simulink model "Vector_control_FOC_with_SVPWM_of_3_phase_induction_motor_drive"  (R2024a)
settings: Solver=ode4  StartTime=0.0  StopTime=3  FixedStep=Ts  MaxStep=1e-4  RelTol=1e-3
PreLoadFcn:
  | Ts=1e-5;
InitFcn:
  | Ts=1e-5;
undefined symbols (not defined in the file): DiscIntNeverNeededParam
libraries: slpidlib x3, spsUniversalBridgeLib x1, spsDCVoltageSourceLib x1, powerlib_extras x1, spsAsynchronousMachineSIUnitsLib x1, simulink x1, spsVoltageMeasurementLib x1, spspowerguiLib x1
Description:
  | Copyright 2011-2013 Ruan Jiayang, Tsinghua Univ.
settings Model: Creator=Hoang Lehuy, Laval University  LastModifiedBy=haris
settings SolverCC: AlgebraicLoopSolver=TrustRegion
settings DataIOCC: SaveFinalState=on  SaveFormat=Array  SignalLoggingSaveFormat=ModelDataLogs  SaveOutput=off  SaveTime=off  ReturnWorkspaceOutputs=off  SignalLoggingName=sigsOut
settings OptimizationCC: BlockReduction=off  ExpressionDepthLimit=2147483647  InitFltsAndDblsToZero=on  LifeSpan=inf
settings DebuggingCC: SaveWithParameterizedLinksMsg=none  UnderspecifiedInitializationDetection=Classic  MergeDetectMultiDrivingBlocksExec=none  CheckExecutionContextPreStartOutputMsg=on  SignalResolutionControl=TryResolveAllWithWarning  MultiTaskDSMMsg=warning  MultiTaskCondExecSysMsg=none  FcnCallInpInsideContextMsg=warning  UnconnectedInputMsg=warning  UnconnectedLineMsg=warning  StateNameClashWarn=warning  SFUnexpectedBacktrackingDiag=warning  SFNoUnconditionalDefaultTransitionDiag=warning  SFExecutionAtInitializationDiag=none  ArithmeticOperatorsInVariantConditions=warning
settings HardwareCC: ProdBitPerPointer=32  ProdBitPerSizeT=32  ProdBitPerPtrDiffT=32  ProdLargestAtomicFloat=None  ProdIntDivRoundTo=Undefined  ProdEndianess=Unspecified  ProdWordSize=32  ProdHWDeviceType=32-bit Generic  TargetUnknown=on
settings ModelReferenceCC: PropagateSignalLabelsOutOfModel=off
settings SFSimCC: SimUseLocalCustomCode=off  SimParseCustomCode=off  CustomCodeUndefinedFunction=UseInterfaceOnly
settings RTWCC: RTWUseLocalCustomCode=off  GPUComputeCapability=3.5
settings CodeAppCC: StateflowObjectComments=on
settings GRTTargetCC: TargetFcnLib=ansi_tfl_tmw.mat  TargetLangStandard=C89/C90 (ANSI)  CombineOutputUpdateFcns=off  GRTInterface=on
settings ConfigComp: CovMetricSettings=dw  CovSaveCumulativeToWorkspaceVar=on  CovSaveSingleToWorkspaceVar=on  CovExternalEMLEnable=off

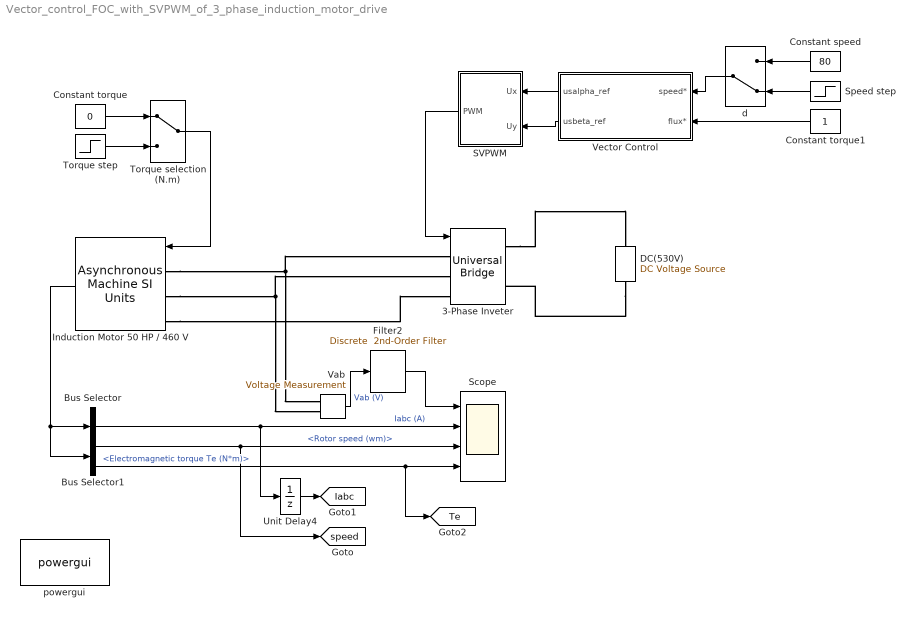
== system Vector_control_FOC_with_SVPWM_of_3_phase_induction_motor_drive ==
  3-Phase Inveter : spsUniversalBridgeLib/Universal Bridge  Arms=3  SnubberResistance=1e5  SnubberCapacitance=1e-6  Device=IGBT / Diodes  Ron=1e-3  Lon=0  ForwardVoltages="[1.1  0.75]"  ForwardVoltage=0  GTOparameters=[ 10e-6 , 20e-6 ]  IGBTparameters=[ 1e-6 , 2e-6 ]  Measurements=None  Measurements_2=None  converterType=Rectifier
  Bus Selector : BusSelector  OutputSignals=Stator measurements.Stator current is_a (A),Stator measurements.Stator current is_b (A),Stator measurements.Stator current is_c (A)  OutputAsBus=on
  Bus Selector1 : BusSelector  OutputSignals=Mechanical.Rotor speed (wm),Mechanical.Electromagnetic torque Te (N*m)
  Constant speed : Constant  Value=80
  Constant torque : Constant  Value=0
  Constant torque1 : Constant
  DC(530V) : spsDCVoltageSourceLib/DC Voltage Source  Amplitude=530  Measurements=None
  Filter2 : powerlib_extras/Discrete  Control Blocks/Discrete  2nd-Order Filter  FilterType=Lowpass  Fo=100  Zeta=0.707  Ts=Ts  Initialize=off  Vac_Init=[0.8 -25 60]  Vdc_Init=-0.4  PlotResponse=off  param1=[1 500 1]
  Induction Motor 50 HP / 460 V : spsAsynchronousMachineSIUnitsLib/Asynchronous Machine SI Units  RotorType=Squirrel-cage  PresetModel=No  MechanicalLoad=Torque Tm  ShowDetailedParameters=on  ReferenceFrame=Stationary  Units=SI  MeasurementBus=off  NominalParameters=[ 50*746, 460, 60 ]  VoltageRatio=1  Stator=[ 0.087 0.8e-3 ]  Rotor="[ 0.228  0.8e-3 ]"  Cage1=[0.4155 0.002066]  Cage2=[0.4168 0.0003495]  Lm=34.7e-3  Mechanical="[1.662  0.01 2 ]"  PolePairs=2  InitialConditions="[ 1, 0 ,  0 , 0 , 0 , 0 , 0 , 0 ]"  SimulateSaturation=off  Saturation=[0 0;0 0]  LoadFlowParameters=0  TsPowergui=0  TsBlock=-1  IterativeModel=Trapezoidal non iterative  IterativeDiscreteModel=Trapezoidal non iterative  Pmec=1.492e+006
      settings: AttributesFormatString=\n
  SVPWM : Subsystem
  Scope : Scope  NumInputPorts=4
  Speed step : Step  Time=1.5  Before=80  After=160  SampleTime=Ts
  Torque selection (N.m) : ManualSwitch
  Torque step : Step  Time=1.8  After=200  SampleTime=0
  Unit Delay4 : UnitDelay  SampleTime=Ts
  Vab : spsVoltageMeasurementLib/Voltage Measurement  Tag=PoWeRsYsTeMmEaSuReMeNt  PhasorSimulation=off  OutputType=Magnitude  PSBequivalent=0
  Vector Control : Subsystem
  d : ManualSwitch  CurrentSetting=0
  powergui : spspowerguiLib/powergui  Priority=2  SimulationMode=Continuous  SampleTime=Ts  frequency=60  Iterations=50  frequencyindice=0  Pbase=100e6  ErrMax=1e-4  UnitsV=kV  UnitsW=MW  buscounter=0  FunctionMessages=off  echomessages=off  EnableUseOfTLC=off  CurrentSourceSwitches=off  DisableSnubberDevices=off  DisableRonSwitches=off  DisableVfSwitches=off  DisplayEquations=off  AutomaticDiscreteSolvers=off  SolverType=Tustin/Backward Euler (TBE)  Interpol=off  ExternalGateDelay=off  methode=off  Ts=0  x0status=blocks  SPID=off  SwTol=0  HookPort=off  NonlinearTolerance=1e-4  nMaxIteration=100  ContinueOnMaxIteration=off  RestoreLinks=warning  ResistiveCurrentMeasurement=off  Frange=[0:2:500]  Ylog=off  Xlog=on  ShowGrid=off  save=off  variable=ZData  structure=0  ZoomFFT=on  StartTime=0.0  cycles=1  DisplayStyle=off  fundamental=60  FreqAxis=off  MaxFrequency=1000  frequencyindicesteady=1  RmsSteady=1  display=off
  tag scope: Iabc=global, Te=global, speed=global
  wires:
  Bus Selector1/1 -> Scope/3, [speed]  "<Rotor speed (wm)>"
  Torque step/1 -> Torque selection (N.m)/2
  Constant torque/1 -> Torque selection (N.m)/1
  Constant speed/1 -> d/1
  Speed step/1 -> d/2
  Bus Selector/1 -> Scope/2, Unit Delay4/1  "Iabc (A)"
  Bus Selector1/2 -> Scope/4, [Te]  "<Electromagnetic torque Te (N*m)>"
  Torque selection (N.m)/1 -> Induction Motor 50 HP / 460 V/1
  Induction Motor 50 HP / 460 V/1 -> Bus Selector1/1, Bus Selector/1
  Unit Delay4/1 -> [Iabc]
  d/1 -> Vector Control/1(speed*)
  Constant torque1/1 -> Vector Control/2(flux*)
  Vector Control/1(usalpha_ref) -> SVPWM/1(Ux)
  Vector Control/2(usbeta_ref) -> SVPWM/2(Uy)
  SVPWM/1(PWM) -> 3-Phase Inveter/1
  Vab/1 -> Filter2/1  "Vab (V)"
  Filter2/1 -> Scope/1
  connections:
  Induction Motor 50 HP / 460 V/LConn2 -- Vab/LConn2 -- 3-Phase Inveter/LConn2
  Induction Motor 50 HP / 460 V/LConn1 -- Vab/LConn1 -- 3-Phase Inveter/LConn1
  Induction Motor 50 HP / 460 V/LConn3 -- 3-Phase Inveter/LConn3
  3-Phase Inveter/RConn1 -- DC(530V)/RConn1
  DC(530V)/LConn1 -- 3-Phase Inveter/RConn2

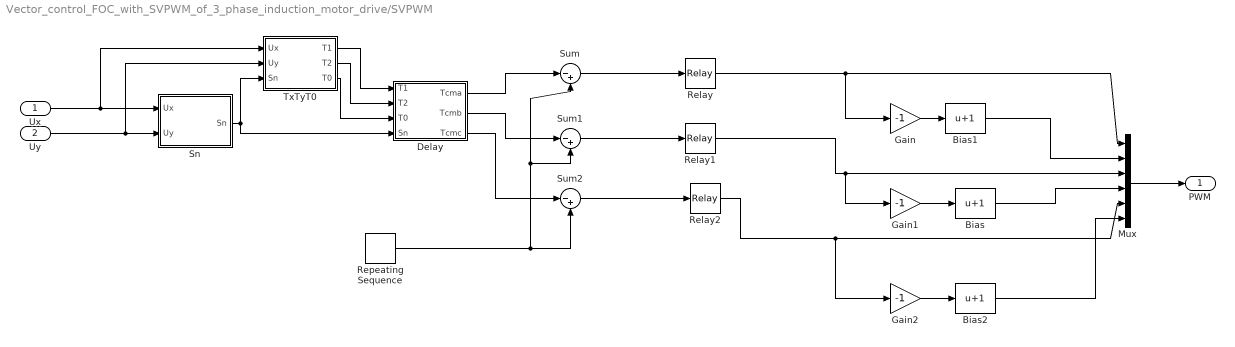
== system Vector_control_FOC_with_SVPWM_of_3_phase_induction_motor_drive/SVPWM ==
  Ux : Inport
  Uy : Inport  Port=2
  Bias : Bias  Bias=1  SaturateOnIntegerOverflow=off
  Bias1 : Bias  Bias=1  SaturateOnIntegerOverflow=off
  Bias2 : Bias  Bias=1  SaturateOnIntegerOverflow=off
  Delay : MATLAB Function  TreatAsAtomicUnit=on
  Gain : Gain  Gain=-1
  Gain1 : Gain  Gain=-1
  Gain2 : Gain  Gain=-1
  Mux : Mux  Inputs=6
  Relay : Relay  OnSwitchValue=0  OffSwitchValue=0
  Relay1 : Relay  OnSwitchValue=0  OffSwitchValue=0
  Relay2 : Relay  OnSwitchValue=0  OffSwitchValue=0
  Repeating Sequence : simulink/Sources/Repeating Sequence  rep_seq_t=[0 1/2000/2 1/2000]  rep_seq_y=[0 1/2000/2 0]
  Sn : MATLAB Function  TreatAsAtomicUnit=on
  Sum : Sum  Inputs=|-+
  Sum1 : Sum  Inputs=|-+
  Sum2 : Sum  Inputs=|-+
  TxTyT0 : MATLAB Function  TreatAsAtomicUnit=on
  PWM : Outport
  wires:
  Delay/1(Tcma) -> Sum/1
  Delay/2(Tcmb) -> Sum1/1
  Delay/3(Tcmc) -> Sum2/1
  Repeating Sequence/1 -> Sum/2, Sum1/2, Sum2/2
  Sum/1 -> Relay/1
  Sum2/1 -> Relay2/1
  Sum1/1 -> Relay1/1
  Relay1/1 -> Mux/3, Gain1/1
  Relay2/1 -> Mux/5, Gain2/1
  Sn/1(Sn) -> TxTyT0/3(Sn), Delay/4(Sn)
  TxTyT0/1(T1) -> Delay/1(T1)
  TxTyT0/2(T2) -> Delay/2(T2)
  TxTyT0/3(T0) -> Delay/3(T0)
  Mux/1 -> PWM/1
  Gain1/1 -> Bias/1
  Gain/1 -> Bias1/1
  Gain2/1 -> Bias2/1
  Bias1/1 -> Mux/2
  Bias/1 -> Mux/4
  Bias2/1 -> Mux/6
  Relay/1 -> Mux/1, Gain/1
  Ux/1 -> Sn/1(Ux), TxTyT0/1(Ux)
  Uy/1 -> Sn/2(Uy), TxTyT0/2(Uy)

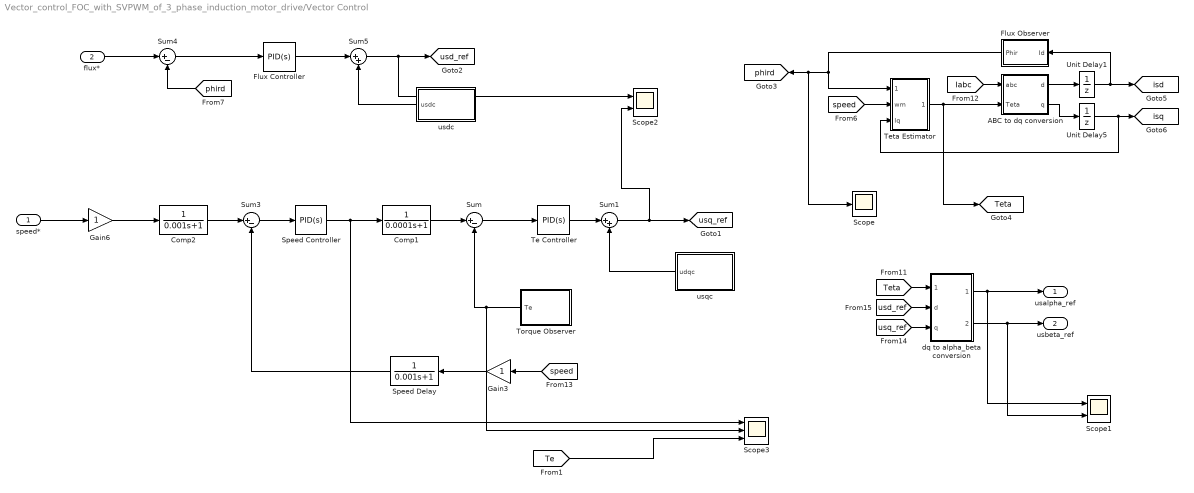
== system Vector_control_FOC_with_SVPWM_of_3_phase_induction_motor_drive/Vector Control ==
  speed* : Inport
  flux* : Inport  Port=2
  ABC to dq conversion : Subsystem
  Comp1 : TransferFcn  Denominator=[0.0001 1]
  Comp2 : TransferFcn  Denominator=[0.001 1]
  Flux Controller : slpidlib/PID Controller  Controller=PID  Form=Parallel  TimeDomain=Continuous-time  UseExternalTs=off  SampleTime=1  IntegratorMethod=Forward Euler  FilterMethod=Forward Euler  ControllerParametersSource=internal  P=138.2107  I=247.3835  UseKiTs=off  D=0  UseExternalDerivativeSource=off  N=100  UseFilter=on  TunerSelectOption=Transfer Function Based (PID Tuner App)  InitialConditionSource=internal  InitialConditionForIntegrator=100  InitialConditionForFilter=0  DifferentiatorICPrevScaledInput=0  ExternalReset=none  TrackingMode=off  Kt=1  LimitOutput=on  SatLimitsSource=internal  UpperSaturationLimit=200  LowerSaturationLimit=-200  LinearizeAsGain=off  AntiWindupMode=clamping  Kb=1  LimitIntegrator=off  UpperIntegratorSaturationLimit=inf  LowerIntegratorSaturationLimit=-inf  POutMin=[]  POutMax=[]  IOutMin=[]  IOutMax=[]  DOutMin=[]  DOutMax=[]  NOutMin=[]  NOutMax=[]  SumOutMin=[]  SumOutMax=[]  SaturationOutMin=[]  SaturationOutMax=[]  PParamMin=[]  PParamMax=[]  IParamMin=[]  IParamMax=[]  DParamMin=[]  DParamMax=[]  NParamMin=[]  NParamMax=[]  KbParamMin=[]  KbParamMax=[]  KtParamMin=[]  KtParamMax=[]  KbOutMin=[]  KbOutMax=[]  KtOutMin=[]  KtOutMax=[]  IntegratorOutMin=[]  IntegratorOutMax=[]  FilterOutMin=[]  FilterOutMax=[]  SumI1OutMin=[]  SumI1OutMax=[]  SumI2OutMin=[]  SumI2OutMax=[]  SumI3OutMin=[]  SumI3OutMax=[]  SumI4OutMin=[]  SumI4OutMax=[]  SumDOutMin=[]  SumDOutMax=[]  DifferentiatorOutMin=[]  DifferentiatorOutMax=[]  FilterDiffOutCoefMin=[]  FilterDiffOutCoefMax=[]  ReciprocalOutMin=[]  ReciprocalOutMax=[]  SumDenOutMin=[]  SumDenOutMax=[]  SumNumOutMin=[]  SumNumOutMax=[]  DivideOutMin=[]  DivideOutMax=[]  UdiffTsProdOutMin=[]  UdiffTsProdOutMax=[]  NTsProdOutMin=[]  NTsProdOutMax=[]  UintegralTsProdOutMin=[]  UintegralTsProdOutMax=[]  UngainTsProdOutMin=[]  UngainTsProdOutMax=[]  ClampingZeroOutDataTypeStr=Inherit: Inherit via back propagation  ClampingZeroOutMin=[]  ClampingZeroOutMax=[]  FilterDenConstantOutDataTypeStr=Inherit: Inherit via back propagation  FilterDenConstantOutMin=[]  FilterDenConstantOutMax=[]  PCopyOutDataTypeStr=Inherit: Inherit via back propagation  PCopyOutMin=[]  PCopyOutMax=[]  NCopyOutDataTypeStr=Inherit: Inherit via back propagation  NCopyOutMin=[]  NCopyOutMax=[]  IntegratorContinuousStateAttributes=''  IntegratorStateMustResolveToSignalObject=off  IntegratorRTWStateStorageClass=Auto  FilterContinuousStateAttributes=''  FilterStateMustResolveToSignalObject=off  FilterRTWStateStorageClass=Auto  ParallelPVariant=InternalParameters  IdealPVariant=Disabled  IVariant=InternalParameters  DVariant=InternalParameters  IntegratorVariant=Continuous  SatVariant=Enabled  AWVariant=ContClampingParallel  PCopyVariant=Disabled  TRVariant=Disabled  FdbkBlocksVariant=Forward  IdealPFdbkVariant=Disabled  SatFdbkVariant=Disabled  DerivativeFilterVariant=ContFilter  NVariant=InternalParameters  NCopyVariant=Disabled  FilterICVariant=InternalICsFilter  IntegratorICVariant=InternalICs  ExternalResetVariant=Disabled  TRSumVariant=Passthrough  SumFdbkVariant=Disabled  SumVariant=Sum_PID  TsampFilterVariant=InternalTs  TsampNgainVariant=Passthrough  TsampIntegralVariant=Disabled_SignalSpec  ExternalSaturationOutDataTypeStr=Inherit: Same as second input  DerivativeSourceVariant=ErrorSignal
  Flux Observer : Subsystem  mask(Flux Calcultation){}
      mask init:
      | NF=0.44572610323020e-6;
      | DF=[1 -0.99998715486734];
  Gain3 : Gain
  Gain6 : Gain
  Scope : Scope
  Scope1 : Scope  NumInputPorts=2
  Scope2 : Scope  NumInputPorts=2
  Scope3 : Scope  NumInputPorts=3
  Speed Controller : slpidlib/PID Controller  Controller=PID  Form=Parallel  TimeDomain=Continuous-time  UseExternalTs=off  SampleTime=1  IntegratorMethod=Forward Euler  FilterMethod=Forward Euler  ControllerParametersSource=internal  P=166.2  I=27700  UseKiTs=off  D=0  UseExternalDerivativeSource=off  N=100  UseFilter=on  TunerSelectOption=Transfer Function Based (PID Tuner App)  InitialConditionSource=internal  InitialConditionForIntegrator=50  InitialConditionForFilter=0  DifferentiatorICPrevScaledInput=0  ExternalReset=none  TrackingMode=off  Kt=1  LimitOutput=on  SatLimitsSource=internal  UpperSaturationLimit=200  LowerSaturationLimit=-200  LinearizeAsGain=off  AntiWindupMode=clamping  Kb=1  LimitIntegrator=off  UpperIntegratorSaturationLimit=inf  LowerIntegratorSaturationLimit=-inf  POutMin=[]  POutMax=[]  IOutMin=[]  IOutMax=[]  DOutMin=[]  DOutMax=[]  NOutMin=[]  NOutMax=[]  SumOutMin=[]  SumOutMax=[]  SaturationOutMin=[]  SaturationOutMax=[]  PParamMin=[]  PParamMax=[]  IParamMin=[]  IParamMax=[]  DParamMin=[]  DParamMax=[]  NParamMin=[]  NParamMax=[]  KbParamMin=[]  KbParamMax=[]  KtParamMin=[]  KtParamMax=[]  KbOutMin=[]  KbOutMax=[]  KtOutMin=[]  KtOutMax=[]  IntegratorOutMin=[]  IntegratorOutMax=[]  FilterOutMin=[]  FilterOutMax=[]  SumI1OutMin=[]  SumI1OutMax=[]  SumI2OutMin=[]  SumI2OutMax=[]  SumI3OutMin=[]  SumI3OutMax=[]  SumI4OutMin=[]  SumI4OutMax=[]  SumDOutMin=[]  SumDOutMax=[]  DifferentiatorOutMin=[]  DifferentiatorOutMax=[]  FilterDiffOutCoefMin=[]  FilterDiffOutCoefMax=[]  ReciprocalOutMin=[]  ReciprocalOutMax=[]  SumDenOutMin=[]  SumDenOutMax=[]  SumNumOutMin=[]  SumNumOutMax=[]  DivideOutMin=[]  DivideOutMax=[]  UdiffTsProdOutMin=[]  UdiffTsProdOutMax=[]  NTsProdOutMin=[]  NTsProdOutMax=[]  UintegralTsProdOutMin=[]  UintegralTsProdOutMax=[]  UngainTsProdOutMin=[]  UngainTsProdOutMax=[]  ClampingZeroOutDataTypeStr=Inherit: Inherit via back propagation  ClampingZeroOutMin=[]  ClampingZeroOutMax=[]  FilterDenConstantOutDataTypeStr=Inherit: Inherit via back propagation  FilterDenConstantOutMin=[]  FilterDenConstantOutMax=[]  PCopyOutDataTypeStr=Inherit: Inherit via back propagation  PCopyOutMin=[]  PCopyOutMax=[]  NCopyOutDataTypeStr=Inherit: Inherit via back propagation  NCopyOutMin=[]  NCopyOutMax=[]  IntegratorContinuousStateAttributes=''  IntegratorStateMustResolveToSignalObject=off  IntegratorRTWStateStorageClass=Auto  FilterContinuousStateAttributes=''  FilterStateMustResolveToSignalObject=off  FilterRTWStateStorageClass=Auto  ParallelPVariant=InternalParameters  IdealPVariant=Disabled  IVariant=InternalParameters  DVariant=InternalParameters  IntegratorVariant=Continuous  SatVariant=Enabled  AWVariant=ContClampingParallel  PCopyVariant=Disabled  TRVariant=Disabled  FdbkBlocksVariant=Forward  IdealPFdbkVariant=Disabled  SatFdbkVariant=Disabled  DerivativeFilterVariant=ContFilter  NVariant=InternalParameters  NCopyVariant=Disabled  FilterICVariant=InternalICsFilter  IntegratorICVariant=InternalICs  ExternalResetVariant=Disabled  TRSumVariant=Passthrough  SumFdbkVariant=Disabled  SumVariant=Sum_PID  TsampFilterVariant=InternalTs  TsampNgainVariant=Passthrough  TsampIntegralVariant=Disabled_SignalSpec  ExternalSaturationOutDataTypeStr=Inherit: Same as second input  DerivativeSourceVariant=ErrorSignal
  Speed Delay : TransferFcn  Denominator=[0.001 1]
  Sum : Sum  Inputs=|+-
  Sum1 : Sum  Inputs=|++
  Sum3 : Sum  Inputs=|+-
  Sum4 : Sum  Inputs=|+-
  Sum5 : Sum  Inputs=|++
  Te Controller : slpidlib/PID Controller  Controller=PID  Form=Parallel  TimeDomain=Continuous-time  UseExternalTs=off  SampleTime=1  IntegratorMethod=Forward Euler  FilterMethod=Forward Euler  ControllerParametersSource=internal  P=2.69732  I=148.34534  UseKiTs=off  D=0  UseExternalDerivativeSource=off  N=100  UseFilter=on  TunerSelectOption=Transfer Function Based (PID Tuner App)  InitialConditionSource=internal  InitialConditionForIntegrator=100  InitialConditionForFilter=0  DifferentiatorICPrevScaledInput=0  ExternalReset=none  TrackingMode=off  Kt=1  LimitOutput=on  SatLimitsSource=internal  UpperSaturationLimit=200  LowerSaturationLimit=-200  LinearizeAsGain=off  AntiWindupMode=clamping  Kb=1  LimitIntegrator=off  UpperIntegratorSaturationLimit=inf  LowerIntegratorSaturationLimit=-inf  POutMin=[]  POutMax=[]  IOutMin=[]  IOutMax=[]  DOutMin=[]  DOutMax=[]  NOutMin=[]  NOutMax=[]  SumOutMin=[]  SumOutMax=[]  SaturationOutMin=[]  SaturationOutMax=[]  PParamMin=[]  PParamMax=[]  IParamMin=[]  IParamMax=[]  DParamMin=[]  DParamMax=[]  NParamMin=[]  NParamMax=[]  KbParamMin=[]  KbParamMax=[]  KtParamMin=[]  KtParamMax=[]  KbOutMin=[]  KbOutMax=[]  KtOutMin=[]  KtOutMax=[]  IntegratorOutMin=[]  IntegratorOutMax=[]  FilterOutMin=[]  FilterOutMax=[]  SumI1OutMin=[]  SumI1OutMax=[]  SumI2OutMin=[]  SumI2OutMax=[]  SumI3OutMin=[]  SumI3OutMax=[]  SumI4OutMin=[]  SumI4OutMax=[]  SumDOutMin=[]  SumDOutMax=[]  DifferentiatorOutMin=[]  DifferentiatorOutMax=[]  FilterDiffOutCoefMin=[]  FilterDiffOutCoefMax=[]  ReciprocalOutMin=[]  ReciprocalOutMax=[]  SumDenOutMin=[]  SumDenOutMax=[]  SumNumOutMin=[]  SumNumOutMax=[]  DivideOutMin=[]  DivideOutMax=[]  UdiffTsProdOutMin=[]  UdiffTsProdOutMax=[]  NTsProdOutMin=[]  NTsProdOutMax=[]  UintegralTsProdOutMin=[]  UintegralTsProdOutMax=[]  UngainTsProdOutMin=[]  UngainTsProdOutMax=[]  ClampingZeroOutDataTypeStr=Inherit: Inherit via back propagation  ClampingZeroOutMin=[]  ClampingZeroOutMax=[]  FilterDenConstantOutDataTypeStr=Inherit: Inherit via back propagation  FilterDenConstantOutMin=[]  FilterDenConstantOutMax=[]  PCopyOutDataTypeStr=Inherit: Inherit via back propagation  PCopyOutMin=[]  PCopyOutMax=[]  NCopyOutDataTypeStr=Inherit: Inherit via back propagation  NCopyOutMin=[]  NCopyOutMax=[]  IntegratorContinuousStateAttributes=''  IntegratorStateMustResolveToSignalObject=off  IntegratorRTWStateStorageClass=Auto  FilterContinuousStateAttributes=''  FilterStateMustResolveToSignalObject=off  FilterRTWStateStorageClass=Auto  ParallelPVariant=InternalParameters  IdealPVariant=Disabled  IVariant=InternalParameters  DVariant=InternalParameters  IntegratorVariant=Continuous  SatVariant=Enabled  AWVariant=ContClampingParallel  PCopyVariant=Disabled  TRVariant=Disabled  FdbkBlocksVariant=Forward  IdealPFdbkVariant=Disabled  SatFdbkVariant=Disabled  DerivativeFilterVariant=ContFilter  NVariant=InternalParameters  NCopyVariant=Disabled  FilterICVariant=InternalICsFilter  IntegratorICVariant=InternalICs  ExternalResetVariant=Disabled  TRSumVariant=Passthrough  SumFdbkVariant=Disabled  SumVariant=Sum_PID  TsampFilterVariant=InternalTs  TsampNgainVariant=Passthrough  TsampIntegralVariant=Disabled_SignalSpec  ExternalSaturationOutDataTypeStr=Inherit: Same as second input  DerivativeSourceVariant=ErrorSignal
  Teta Estimator : Subsystem
  Torque Observer : Subsystem
  Unit Delay1 : UnitDelay  SampleTime=Ts
  Unit Delay5 : UnitDelay  SampleTime=Ts
  dq to alpha_beta conversion : Subsystem
  usdc : Subsystem
  usqc : Subsystem
  usalpha_ref : Outport
  usbeta_ref : Outport  Port=2
  tag scope: Teta=global, isd=global, isq=global, phird=global, usd_ref=global, usq_ref=global
  wires:
  Sum/1 -> Te Controller/1
  Comp1/1 -> Sum/1
  Te Controller/1 -> Sum1/1
  usqc/1(udqc) -> Sum1/2
  Torque Observer/1(Te) -> Sum/2, Scope3/2
  Sum1/1 -> [usq_ref], Scope2/2
  [speed] -> Gain3/1
  Sum3/1 -> Speed Controller/1
  Gain3/1 -> Speed Delay/1
  Comp2/1 -> Sum3/1
  flux*/1 -> Sum4/1
  [phird] -> Sum4/2
  Sum4/1 -> Flux Controller/1
  Flux Controller/1 -> Sum5/1
  Sum5/1 -> [usd_ref], Scope2/1
  Flux Observer/1(Phir) -> Teta Estimator/1(Phird), [phird], Scope/1
  Teta Estimator/1(Teta) -> ABC to dq conversion/2(Teta), [Teta]
  [speed] -> Teta Estimator/2(wm)
  [Iabc] -> ABC to dq conversion/1(abc)
  [Teta] -> dq to alpha_beta conversion/1(Teta)
  Gain6/1 -> Comp2/1
  speed*/1 -> Gain6/1
  ABC to dq conversion/1(d) -> Unit Delay1/1
  Unit Delay1/1 -> [isd], Flux Observer/1(Id)
  ABC to dq conversion/2(q) -> Unit Delay5/1
  Unit Delay5/1 -> Teta Estimator/3(Iq), [isq]
  [usd_ref] -> dq to alpha_beta conversion/2(d)
  [usq_ref] -> dq to alpha_beta conversion/3(q)
  usdc/1(usdc) -> Sum5/2
  Speed Delay/1 -> Sum3/2
  Speed Controller/1 -> Comp1/1, Scope3/1
  [Te] -> Scope3/3
  dq to alpha_beta conversion/1(usalpha) -> usalpha_ref/1, Scope1/1
  dq to alpha_beta conversion/2(usbeta) -> usbeta_ref/1, Scope1/2

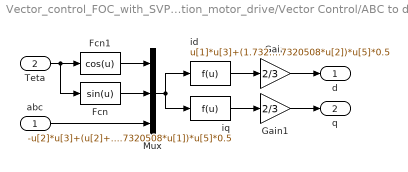
== system Vector_control_FOC_with_SVPWM_of_3_phase_induction_motor_drive/Vector Control/ABC to dq conversion ==
  abc : Inport
  Teta : Inport  Port=2
  Fcn : Fcn  Expr=sin(u)
  Fcn1 : Fcn  Expr=cos(u)
  Gain : Gain  Gain=2/3  SaturateOnIntegerOverflow=on  OutDataTypeStr=Inherit: Same as input  ParamDataTypeStr=Inherit: Same as input
  Gain1 : Gain  Gain=2/3  SaturateOnIntegerOverflow=on  OutDataTypeStr=Inherit: Same as input  ParamDataTypeStr=Inherit: Same as input
  Mux : Mux  Inputs=[1 1 3]
  id : Fcn  Expr=u[1]*u[3]+(1.7320508*u[2]-u[1])*u[4]*0.5+(-u[1]-1.7320508*u[2])*u[5]*0.5
  iq : Fcn  Expr=-u[2]*u[3]+(u[2]+1.7320508*u[1])*u[4]*0.5+(u[2]-1.7320508*u[1])*u[5]*0.5
  d : Outport  InitialOutput=0
  q : Outport  Port=2  InitialOutput=0
  wires:
  Fcn/1 -> Mux/2
  Fcn1/1 -> Mux/1
  Teta/1 -> Fcn1/1, Fcn/1
  Mux/1 -> iq/1, id/1
  abc/1 -> Mux/3
  iq/1 -> Gain1/1
  id/1 -> Gain/1
  Gain/1 -> d/1
  Gain1/1 -> q/1

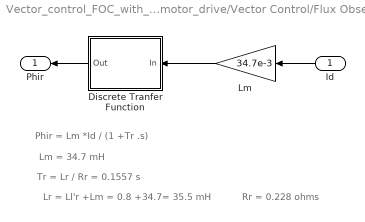
== system Vector_control_FOC_with_SVPWM_of_3_phase_induction_motor_drive/Vector Control/Flux Observer ==
  note: Phir = Lm *Id / (1 +Tr .s)
  note: Lm = 34.7 mH
  note: Lr = Ll'r +Lm = 0.8 +34.7= 35.5 mH
  note: Tr = Lr / Rr = 0.1557 s
  note: Rr = 0.228 ohms
  Id : Inport
  Discrete Tranfer Function : Subsystem  mask(First Order Low Pass Filter (Discrete)){T=0.1557, Ts=Ts}
      mask prompts: T "Time constant T (s) :"; Ts "Time step (s)"
      mask help: H(s)=1/(1+T.s)
      mask init:
      | X=[0 1 2 3 4];
      |  Y=[-2 -2 -3 -4 -4];
      |  str=sprintf('\nH=1/(1+T.s)\n T= %g s\n\n\n',T);
      | num=1;
      | den=[T 1];
      | 
      | % discrete transfer function
      | % descending powers of z
      | numd= Ts/T;
      | dend=[ 1  (Ts-T)/T];
      mask Display:
      | plot(X,Y);
      | disp(str);
  Lm : Gain  Gain=34.7e-3  SaturateOnIntegerOverflow=on  OutDataTypeStr=Inherit: Same as input  ParamDataTypeStr=Inherit: Same as input
  Phir : Outport
  wires:
  Discrete Tranfer Function/1(Out) -> Phir/1
  Id/1 -> Lm/1
  Lm/1 -> Discrete Tranfer Function/1(In)

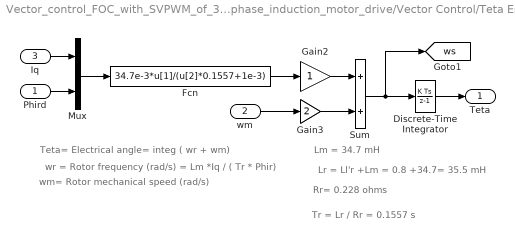
== system Vector_control_FOC_with_SVPWM_of_3_phase_induction_motor_drive/Vector Control/Teta Estimator ==
  note: Teta= Electrical angle= integ ( wr + wm)
  note: wr = Rotor frequency (rad/s) = Lm *Iq / ( Tr * Phir)
  note: Lm = 34.7 mH
  note: Rr= 0.228 ohms
  note: Lr = Ll'r +Lm = 0.8 +34.7= 35.5 mH
  note: wm= Rotor mechanical speed (rad/s)
  note: Tr = Lr / Rr = 0.1557 s
  Phird : Inport
  wm : Inport  Port=2
  Iq : Inport  Port=3
  Discrete-Time Integrator : DiscreteIntegrator  SampleTime=Ts  ICPrevOutput=DiscIntNeverNeededParam  ICPrevScaledInput=DiscIntNeverNeededParam
  Fcn : Fcn  Expr=34.7e-3*u[1]/(u[2]*0.1557+1e-3)
  Gain2 : Gain  SaturateOnIntegerOverflow=on  OutDataTypeStr=Inherit: Same as input  ParamDataTypeStr=Inherit: Same as input
  Gain3 : Gain  Gain=2  SaturateOnIntegerOverflow=on  OutDataTypeStr=Inherit: Same as input  ParamDataTypeStr=Inherit: Same as input
  Mux : Mux  Inputs=2
  Sum : Sum  InputSameDT=on  SaturateOnIntegerOverflow=on  OutDataTypeStr=Inherit: Same as first input
  Teta : Outport  InitialOutput=0
  tag scope: ws=global
  wires:
  Discrete-Time Integrator/1 -> Teta/1
  Sum/1 -> Discrete-Time Integrator/1, [ws]
  Gain3/1 -> Sum/2
  Gain2/1 -> Sum/1
  wm/1 -> Gain3/1
  Fcn/1 -> Gain2/1
  Phird/1 -> Mux/2
  Iq/1 -> Mux/1
  Mux/1 -> Fcn/1

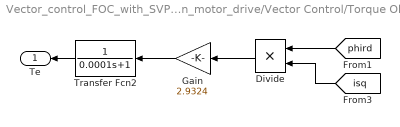
== system Vector_control_FOC_with_SVPWM_of_3_phase_induction_motor_drive/Vector Control/Torque Observer ==
  Divide : Product
  Gain : Gain  Gain=2.9324
  Transfer Fcn2 : TransferFcn  Denominator=[0.0001 1]
  Te : Outport
  wires:
  [phird] -> Divide/1
  Divide/1 -> Gain/1
  Gain/1 -> Transfer Fcn2/1
  [isq] -> Divide/2
  Transfer Fcn2/1 -> Te/1

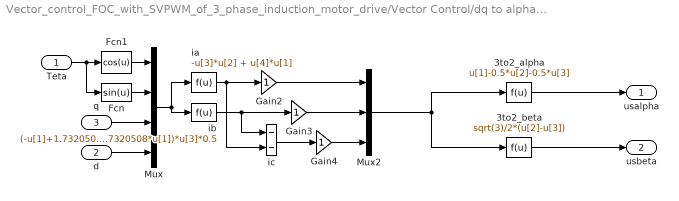
== system Vector_control_FOC_with_SVPWM_of_3_phase_induction_motor_drive/Vector Control/dq to alpha_beta conversion ==
  Teta : Inport
  d : Inport  Port=2
  q : Inport  Port=3
  3to2_alpha : Fcn  Expr=u[1]-0.5*u[2]-0.5*u[3]
  3to2_beta : Fcn  Expr=sqrt(3)/2*(u[2]-u[3])
  Fcn : Fcn  Expr=sin(u)
  Fcn1 : Fcn  Expr=cos(u)
  Gain2 : Gain  SaturateOnIntegerOverflow=on  OutDataTypeStr=Inherit: Same as input  ParamDataTypeStr=Inherit: Same as input
  Gain3 : Gain  SaturateOnIntegerOverflow=on  OutDataTypeStr=Inherit: Same as input  ParamDataTypeStr=Inherit: Same as input
  Gain4 : Gain  SaturateOnIntegerOverflow=on  OutDataTypeStr=Inherit: Same as input  ParamDataTypeStr=Inherit: Same as input
  Mux : Mux
  Mux2 : Mux  Inputs=3
  ia : Fcn  Expr=-u[3]*u[2] + u[4]*u[1]
  ib : Fcn  Expr=(-u[1]+1.7320508*u[2])*u[4]*0.5+(u[2]+1.7320508*u[1])*u[3]*0.5
  ic : Sum  Inputs=--  InputSameDT=on  SaturateOnIntegerOverflow=on  OutDataTypeStr=Inherit: Same as first input
  usalpha : Outport
  usbeta : Outport  Port=2
  wires:
  Fcn/1 -> Mux/2
  Fcn1/1 -> Mux/1
  Mux/1 -> ib/1, ia/1
  Teta/1 -> Fcn1/1, Fcn/1
  q/1 -> Mux/3
  d/1 -> Mux/4
  Gain3/1 -> Mux2/2
  ic/1 -> Gain4/1
  Gain4/1 -> Mux2/3
  Gain2/1 -> Mux2/1
  ia/1 -> Gain2/1, ic/2
  ib/1 -> Gain3/1, ic/1
  Mux2/1 -> 3to2_alpha/1, 3to2_beta/1
  3to2_alpha/1 -> usalpha/1
  3to2_beta/1 -> usbeta/1

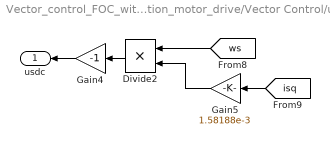
== system Vector_control_FOC_with_SVPWM_of_3_phase_induction_motor_drive/Vector Control/usdc ==
  Divide2 : Product
  Gain4 : Gain  Gain=-1
  Gain5 : Gain  Gain=1.58188e-3
  usdc : Outport
  wires:
  Divide2/1 -> Gain4/1
  [ws] -> Divide2/1
  [isq] -> Gain5/1
  Gain5/1 -> Divide2/2
  Gain4/1 -> usdc/1

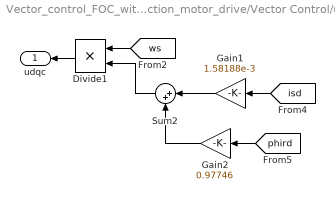
== system Vector_control_FOC_with_SVPWM_of_3_phase_induction_motor_drive/Vector Control/usqc ==
  Divide1 : Product
  Gain1 : Gain  Gain=1.58188e-3
  Gain2 : Gain  Gain=0.97746
  Sum2 : Sum  Inputs=|++
  udqc : Outport
  wires:
  [ws] -> Divide1/1
  Sum2/1 -> Divide1/2
  Gain1/1 -> Sum2/1
  Gain2/1 -> Sum2/2
  [isd] -> Gain1/1
  [phird] -> Gain2/1
  Divide1/1 -> udqc/1

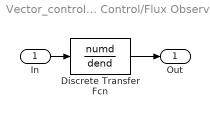
== system Vector_control_FOC_with_SVPWM_of_3_phase_induction_motor_drive/Vector Control/Flux Observer/Discrete Tranfer Function ==
  In : Inport
  Discrete Transfer Fcn : DiscreteTransferFcn  Numerator=numd  Denominator=dend  SampleTime=Ts
  Out : Outport  InitialOutput=0
  wires:
  Discrete Transfer Fcn/1 -> Out/1
  In/1 -> Discrete Transfer Fcn/1

== matlab function Vector_control_FOC_with_SVPWM_of_3_phase_induction_motor_drive/SVPWM/Sn ==
  data: Sn output; Ux input; Uy input
function Sn = S(Ux,Uy)
theta=atan2(Uy,Ux)*180/pi;
if theta>=0&&theta<60
    Sn=1;
elseif theta>=60&&theta<120
    Sn=2;
elseif theta>=120&&theta<180
    Sn=3;
elseif theta>=-180&&theta<-120
    Sn=4;
elseif theta>=-120&&theta<-60
    Sn=5;
else Sn=6;
end

== matlab function Vector_control_FOC_with_SVPWM_of_3_phase_induction_motor_drive/SVPWM/TxTyT0 ==
  data: Ux input; Uy input; Sn input; T1 output; T2 output; T0 output
function [T1,T2,T0]=T(Ux,Uy,Sn)
Ts=1/2000;
Udc=530;

X=sqrt(3)*Ts/Udc*Uy;
Y=sqrt(3)*Ts/2/Udc*(sqrt(3)*Ux+Uy);
Z=sqrt(3)*Ts/2/Udc*(-sqrt(3)*Ux+Uy);

if Sn==1
    T1=-Z;T2=X;
elseif Sn==2;
    T1=Z;T2=Y;
elseif Sn==3;
    T1=X;T2=-Y;
elseif Sn==4;
    T1=-X;T2=Z;
elseif Sn==5;
    T1=-Y;T2=-Z;
else T1=Y;T2=-X;
end
    
if T1+T2>Ts
    a=T1;b=T2;
    T1=a*Ts/(a+b);
    T2=b*Ts/(a+b);
end

T0=Ts-T1-T2;

== matlab function Vector_control_FOC_with_SVPWM_of_3_phase_induction_motor_drive/SVPWM/Delay ==
  data: T1 input; T2 input; T0 input; Tcma output; Tcmb output; Tcmc output; Sn input
function [Tcma,Tcmb,Tcmc]=D(T1,T2,T0,Sn)
T=1/2000;
Udc=530;
ton1=0.25*T0;
ton2=ton1+T1/2;
ton3=ton2+T2/2;
if Sn==1
    Tcma=ton1;Tcmb=ton2;Tcmc=ton3;
elseif Sn==2;
    Tcma=ton2;Tcmb=ton1;Tcmc=ton3;
elseif Sn==3;
    Tcma=ton3;Tcmb=ton1;Tcmc=ton2;
elseif Sn==4;
    Tcma=ton3;Tcmb=ton2;Tcmc=ton1;
elseif Sn==5;
    Tcma=ton2;Tcmb=ton3;Tcmc=ton1;
else Tcma=ton1;Tcmb=ton3;Tcmc=ton2;
end
